simulink model "Admittance_Testbench"  (R2025b)
settings: Solver=ode4  StartTime=0.0  StopTime=inf  FixedStep=0.0005  RelTol=1e-3
undefined symbols (not defined in the file): Ts
settings Model: Creator=Compu  LastModifiedBy=Compu

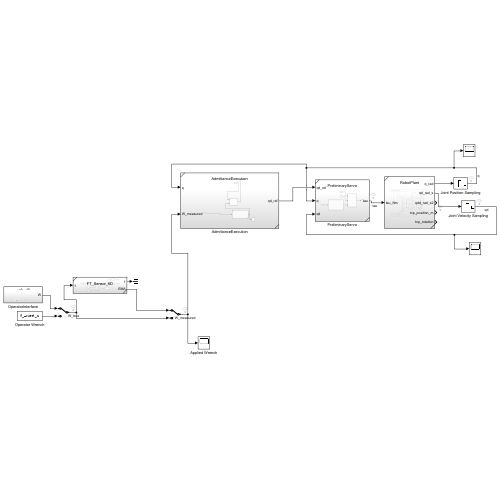
[thumbnail: Simulink's stored preview of the top-level diagram]
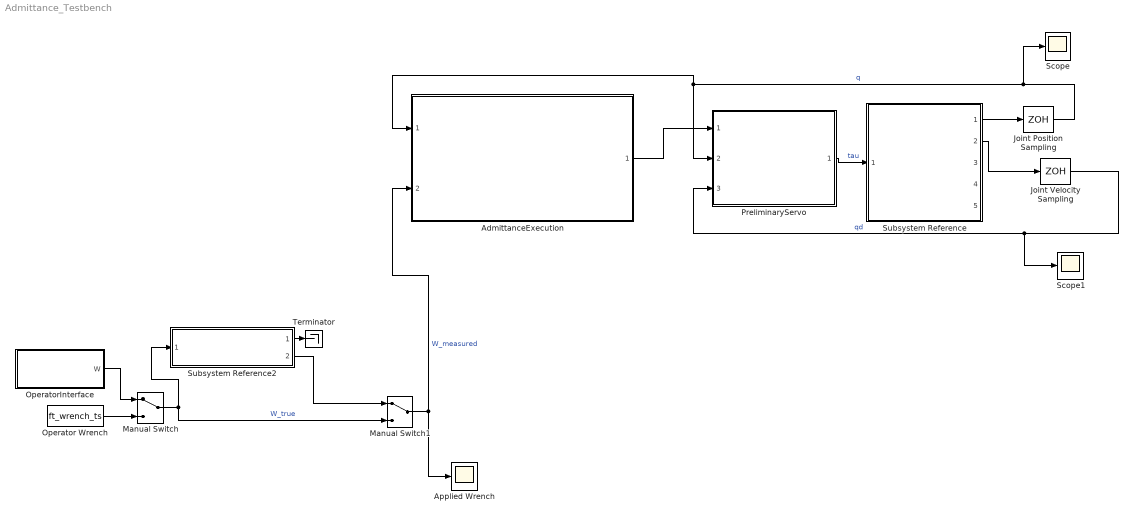
== system Admittance_Testbench ==
  AdmittanceExecution : Subsystem  ReferencedSubsystem=AdmittanceExecution
  Applied Wrench : Scope
      settings: DataLoggingVariableName=ScopeData3
  Joint Position Sampling : ZeroOrderHold  SampleTime=Ts
  Joint Velocity Sampling : ZeroOrderHold  SampleTime=Ts
  Manual Switch : ManualSwitch
  Manual Switch1 : ManualSwitch
  Operator Wrench : FromWorkspace  VariableName=ft_wrench_ts  SampleTime=Ts  Interpolate=off  OutputAfterFinalValue=Holding final value
  OperatorInterface : Subsystem
  PreliminaryServo : Subsystem  ReferencedSubsystem=PreliminaryServo
  Scope : Scope
      settings: ActiveDisplayYMinimum=-2.6907831524345722  ActiveDisplayYMaximum=2.8517336165082168
  Scope1 : Scope
      settings: ActiveDisplayYMinimum=-1  ActiveDisplayYMaximum=1  DataLoggingVariableName=ScopeData2
  Subsystem Reference : Subsystem  ReferencedSubsystem=RobotPlant
  Subsystem Reference2 : Subsystem  ReferencedSubsystem=FT_Sensor_6D
  Terminator : Terminator
  wires:
  Subsystem Reference/1 -> Joint Position Sampling/1
  Subsystem Reference/2 -> Joint Velocity Sampling/1
  Joint Position Sampling/1 -> Scope/1, PreliminaryServo/2, AdmittanceExecution/1  "q"
  Joint Velocity Sampling/1 -> Scope1/1, PreliminaryServo/3  "qd"
  PreliminaryServo/1 -> Subsystem Reference/1  "tau"
  Operator Wrench/1 -> Manual Switch/2
  OperatorInterface/1(W) -> Manual Switch/1
  Manual Switch1/1 -> Applied Wrench/1, AdmittanceExecution/2  "W_measured"
  Manual Switch/1 -> Manual Switch1/2, Subsystem Reference2/1  "W_true"
  Subsystem Reference2/2 -> Manual Switch1/1
  Subsystem Reference2/1 -> Terminator/1
  AdmittanceExecution/1 -> PreliminaryServo/1

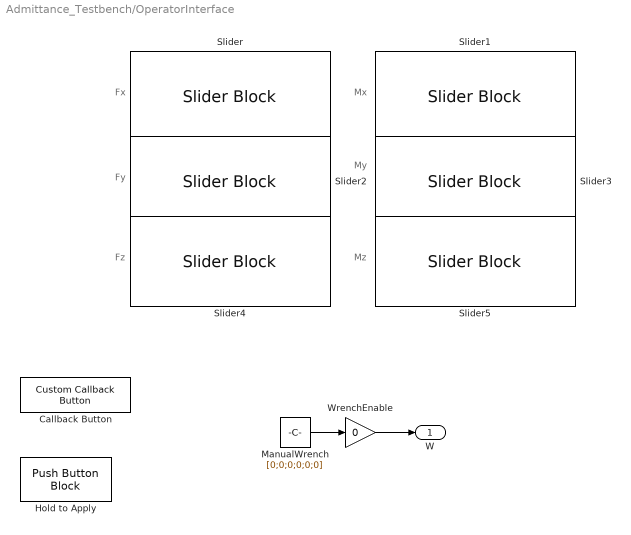
== system Admittance_Testbench/OperatorInterface ==
  note: Fx
  note: Fy
  note: Fz
  note: Mx
  note: My
  note: Mz
  Callback Button : CustomCallbackButton  Configuration="{\"components\":[{\"name\":\"BackgroundImageComponent\",\"settings\":{\"image\":{\"size\":[0,0],\"src\":\"default\",\"srcOrientation\":\"Right\"},\"position\":[0,0,1,1]}},{\"name\":\"ButtonStateComponent\",\"settings\":{\"buttonType\":\"momentary\",\"clickFcn\":\"set_param('Admittance_Testbench\\/OperatorInterface\\/ManualWrench', ...\\n          'Value', '[0;0;0;0;0;0]');\",\"onValue\":1,\"position\":[0,0,1,1],\"pressDelay\":\"500\",\"pressFcn\":\"\",\"repeatInterval\":\"0\",\"states\":[{\"horizontalAlignment\":\"center\",\"image\":{\"position\":[0,0,1,1],\"size\":[1,1],\"src\":\"default\",\"srcOrientation\":\"Right\"},\"label\":{\"color\":[0.01176470588,0.01176470588,0.01176470588,1],\"icon\":{\"size\":[0,0],\"src\":\"default\",\"srcOrientation\":\"Right\"},\"iconOffset\":0,\"iconPlacement\":\"left\",\"opacity\":1,\"show\":true,\"text\":{\"content\":\"Reset All\",\"font\":\"Helvetica\"}},\"labelOffset\":[0,0],\"verticalAlignment\":\"middle\"},{\"horizontalAlignment\":\"center\",\"image\":{\"position\":[0,0,1,1],\"size\":[1,1],\"src\":\"default\",\"srcOrientation\":\"Right\"},\"label\":{\"color\":[0.01176470588,0.01176470588,0.01176470588,1],\"icon\":{\"size\":[0,0],\"src\":\"default\",\"srcOrientation\":\"Right\"},\"iconOffset\":0,\"iconPlacement\":\"left\",\"opacity\":1,\"show\":true,\"text\":{\"content\":\"Reset All\",\"font\":\"Helvetica\"}},\"labelOffset\":[0,0],\"verticalAlignment\":\"middle\"},{\"horizontalAlignment\":\"center\",\"image\":{\"position\":[0,0,1,1],\"size\":[1,1],\"src\":\"default\",\"srcOrientation\":\"Right\"},\"label\":{\"color\":[0.01176470588,0.01176470588,0.01176470588,1],\"icon\":{\"size\":[0,0],\"src\":\"default\",\"srcOrientation\":\"Right\"},\"iconOffset\":0,\"iconPlacement\":\"left\",\"opacity\":1,\"show\":true,\"text\":{\"content\":\"Reset All\",\"font\":\"Helvetica\"}},\"labelOffset\":[0,0],\"verticalAlignment\":\"middle\"},{\"horizontalAlignment\":\"center\",\"image\":{\"position\":[0,0,1,1],\"size\":[1,1],\"src\":\"default\",\"srcOrientation\":\"Right\"},\"label\":{\"color\":[0.01176470588,0.01176470588,0.01176470588,1],\"icon\":{\"size\":[0,0],\"src\":\"default\",\"srcOrientation\":\"Right\"},\"iconOffset\":0,\"iconPlacement\":\"left\",\"opacity\":1,\"show\":true,\"text\":{\"content\":\"Reset All\",\"font\":\"Helvetica\"}},\"labelOffset\":[0,0],\"verticalAlignment\":\"middle\"}]}},{\"name\":\"ForegroundImageComponent\",\"settings\":{\"image\":{\"size\":[0,0],\"src\":\"default\",\"srcOrientation\":\"Right\"},\"isForeground\":1,\"position\":[0,0,1,1]}}],\"derived\":{\"blockParameters\":{\"AutoActivate\":true,\"ButtonText\":\"Reset All\",\"ButtonType\":\"Momentary\",\"ClickFcn\":\"set_param('Admittance_Testbench\\/OperatorInterface\\/ManualWrench', ...\\n          'Value', '[0;0;0;0;0;0]');\",\"OnValue\":1,\"PressDelay\":\"500\",\"PressFcn\":\"\",\"RepeatInterval\":\"0\",\"fixedAspectRatio\":\"off\"}},\"settings\":{\"BindingType\":\"standalone\",\"autoActivate\":true,\"backgroundColor\":[244,244,244,1],\"backgroundOffset\":0.2,\"backgroundOpacity\":1,\"fixedAspectRatio\":\"off\",\"foregroundColor\":[0.01176470588,0.01176470588,0.01176470588,1],\"migratedFromLegacy\":true,\"useBackgroundColor\":true,\"variant\":\"callback\",\"version\":\"R2025a\"},\"type\":\"Button\"}"  CustomBackgroundColor="{\"color\":[0.9568627451,0.9568627451,0.9568627451],\"show\":true}"
  Hold to Apply : PushButtonBlock  ButtonText=Hold to Apply  IconOnColor=[0.0, 0.39215686274509803, 0.0]  IconOffColor=[0.0, 1.0, 0.0]  OffValue=0.000000
  ManualWrench : Constant  Value=[0;0;0;0;0;0]  SampleTime=Ts
  Slider : SliderBlock  ScaleMin=-10  ScaleMax=10  TickInterval=5
  Slider1 : SliderBlock  ScaleMin=-1  ScaleMax=1  TickInterval=0.5
  Slider2 : SliderBlock  ScaleMin=-10  ScaleMax=10  TickInterval=5
  Slider3 : SliderBlock  ScaleMin=-1  ScaleMax=1  TickInterval=0.5
  Slider4 : SliderBlock  ScaleMin=-10  ScaleMax=10  TickInterval=5
  Slider5 : SliderBlock  ScaleMin=-1  ScaleMax=1  TickInterval=0.5
  WrenchEnable : Gain  Gain=0
  W : Outport
  wires:
  ManualWrench/1 -> WrenchEnable/1
  WrenchEnable/1 -> W/1
